simulink model "sm_car_"  (R2026b)
settings: Solver=ode23t  StopTime=100  MaxStep=0.4  AbsTol=1e-3  EnableMultiTasking=on
PreLoadFcn:
  | % Due to usability issue in Repeating Sequence block
  | warning('off','Simulink:Masking:Invalid');
  | 
  | % Eliminate unnecessary warnings in inactive variants
  | % Warnings generated only if you click through inactive variant
  | warning('off','MATLAB:nonExistentField');
  | warning('off','Simulink:Parameters:BlkParamUndefined');
PostLoadFcn:
  | set_param([bdroot '/Vehicle'],'popup_trailer','Off')
  | warning('off','sm:sli:setup:compile:LocalSolverNotSupported')
  | %sm_car_config_maneuver(bdroot,'WOT Braking');
  | sm_car_config_vehicle(bdroot,'false');
  | sm_car_config_logging(bdroot);
InitFcn:
  | sm_car_config_camera;
  | Vehicle = sm_car_vehcfg_checkConfig(Vehicle);
  | sm_car_check_tire_model(bdroot);
StartFcn:
  | tic;
StopFcn:
  | Elapsed_Sim_Time = toc;
  | % disp(['Elapsed Sim Time = ' num2str(Elapsed_Sim_Time)]);
undefined symbols (not defined in the file or in its folder): acc_theta, accel_ramp_rate, Axle1D, AxleIn, Camera, Control, Driver, Init, Maneuver, Pedal, Scene, ShaftL1, ShaftL2, ShaftR1, ShaftR2, Visual, X, xy_data_car_side, Y, Z
libraries: sm_lib x290, fl_lib x171, nesl_utility x144, simulink x60, simulink_extras x14, sdl_lib x14, SimscapeFluids_lib x7, Damper_Element x4, Tire_1x2x x4, ee_lib x3, Scene_Utilities x3, sharedTrackingLibrary x2
(part 3 of 22)

== system sm_car_/Camera Frames/Transform FR ==
  Transform Camera Frame : sm_lib/Frames and Transforms/Rigid Transform  RotationMethod=RotationSequence  FollAlignAxisA=+X  BaseAlignAxisA=+Y  FollAlignAxisB=+Y  BaseAlignAxisB=+Z  RotationStandardAxis=+Z  RotationAngle=0.0  RotationAngleUnits=deg  RotationArbitraryAxis=[0 0 1]  RotationSequenceAxes=FollowerAxes  RotationSequence=ZYX  RotationSequenceAngles=CF.a.Value(3:-1:1)  RotationSequenceAnglesUnits=deg  RotationMatrix=[1 0 0; 0 1 0; 0 0 1]  Quaternion=[1 0 0 0]  TranslationMethod=Cartesian  TranslationCartesianOffset=CF.s.Value  TranslationCartesianOffsetUnits=m  TranslationStandardAxis=+Z  TranslationStandardOffset=0  TranslationStandardOffsetUnits=m  TranslationROffset=0  TranslationROffsetUnits=m  TranslationThetaOffset=0  TranslationThetaOffsetUnits=deg  TranslationZOffset=0  TranslationZOffsetUnits=m
  B : PMIOPort  Side=Left
  F : PMIOPort  Port=2  Side=Right
  connections:
  Transform Camera Frame/RConn1 -- F/RConn1
  Transform Camera Frame/LConn1 -- B/RConn1

== system sm_car_/Camera Frames/Transform FixO FL ==
  Transform Camera Frame : sm_lib/Frames and Transforms/Rigid Transform  RotationMethod=RotationSequence  FollAlignAxisA=+X  BaseAlignAxisA=+Y  FollAlignAxisB=+Y  BaseAlignAxisB=+Z  RotationStandardAxis=+Z  RotationAngle=0.0  RotationAngleUnits=deg  RotationArbitraryAxis=[0 0 1]  RotationSequenceAxes=FollowerAxes  RotationSequence=ZYX  RotationSequenceAngles=CF.a.Value(3:-1:1)  RotationSequenceAnglesUnits=deg  RotationMatrix=[1 0 0; 0 1 0; 0 0 1]  Quaternion=[1 0 0 0]  TranslationMethod=Cartesian  TranslationCartesianOffset=CF.s.Value  TranslationCartesianOffsetUnits=m  TranslationStandardAxis=+Z  TranslationStandardOffset=0  TranslationStandardOffsetUnits=m  TranslationROffset=0  TranslationROffsetUnits=m  TranslationThetaOffset=0  TranslationThetaOffsetUnits=deg  TranslationZOffset=0  TranslationZOffsetUnits=m
  B : PMIOPort  Side=Left
  F : PMIOPort  Port=2  Side=Right
  connections:
  Transform Camera Frame/RConn1 -- F/RConn1
  Transform Camera Frame/LConn1 -- B/RConn1

== system sm_car_/Camera Frames/Transform FixO FR ==
  Transform Camera Frame : sm_lib/Frames and Transforms/Rigid Transform  RotationMethod=RotationSequence  FollAlignAxisA=+X  BaseAlignAxisA=+Y  FollAlignAxisB=+Y  BaseAlignAxisB=+Z  RotationStandardAxis=+Z  RotationAngle=0.0  RotationAngleUnits=deg  RotationArbitraryAxis=[0 0 1]  RotationSequenceAxes=FollowerAxes  RotationSequence=ZYX  RotationSequenceAngles=CF.a.Value(3:-1:1)  RotationSequenceAnglesUnits=deg  RotationMatrix=[1 0 0; 0 1 0; 0 0 1]  Quaternion=[1 0 0 0]  TranslationMethod=Cartesian  TranslationCartesianOffset=CF.s.Value  TranslationCartesianOffsetUnits=m  TranslationStandardAxis=+Z  TranslationStandardOffset=0  TranslationStandardOffsetUnits=m  TranslationROffset=0  TranslationROffsetUnits=m  TranslationThetaOffset=0  TranslationThetaOffsetUnits=deg  TranslationZOffset=0  TranslationZOffsetUnits=m
  B : PMIOPort  Side=Left
  F : PMIOPort  Port=2  Side=Right
  connections:
  Transform Camera Frame/RConn1 -- F/RConn1
  Transform Camera Frame/LConn1 -- B/RConn1

== system sm_car_/Camera Frames/Transform FixO Front ==
  Transform Camera Frame : sm_lib/Frames and Transforms/Rigid Transform  RotationMethod=RotationSequence  FollAlignAxisA=+X  BaseAlignAxisA=+Y  FollAlignAxisB=+Y  BaseAlignAxisB=+Z  RotationStandardAxis=+Z  RotationAngle=0.0  RotationAngleUnits=deg  RotationArbitraryAxis=[0 0 1]  RotationSequenceAxes=FollowerAxes  RotationSequence=ZYX  RotationSequenceAngles=CF.a.Value(3:-1:1)  RotationSequenceAnglesUnits=deg  RotationMatrix=[1 0 0; 0 1 0; 0 0 1]  Quaternion=[1 0 0 0]  TranslationMethod=Cartesian  TranslationCartesianOffset=CF.s.Value  TranslationCartesianOffsetUnits=m  TranslationStandardAxis=+Z  TranslationStandardOffset=0  TranslationStandardOffsetUnits=m  TranslationROffset=0  TranslationROffsetUnits=m  TranslationThetaOffset=0  TranslationThetaOffsetUnits=deg  TranslationZOffset=0  TranslationZOffsetUnits=m
  B : PMIOPort  Side=Left
  F : PMIOPort  Port=2  Side=Right
  connections:
  Transform Camera Frame/RConn1 -- F/RConn1
  Transform Camera Frame/LConn1 -- B/RConn1

== system sm_car_/Camera Frames/Transform FixO Left ==
  Transform Camera Frame : sm_lib/Frames and Transforms/Rigid Transform  RotationMethod=RotationSequence  FollAlignAxisA=+X  BaseAlignAxisA=+Y  FollAlignAxisB=+Y  BaseAlignAxisB=+Z  RotationStandardAxis=+Z  RotationAngle=0.0  RotationAngleUnits=deg  RotationArbitraryAxis=[0 0 1]  RotationSequenceAxes=FollowerAxes  RotationSequence=ZYX  RotationSequenceAngles=CF.a.Value(3:-1:1)  RotationSequenceAnglesUnits=deg  RotationMatrix=[1 0 0; 0 1 0; 0 0 1]  Quaternion=[1 0 0 0]  TranslationMethod=Cartesian  TranslationCartesianOffset=CF.s.Value  TranslationCartesianOffsetUnits=m  TranslationStandardAxis=+Z  TranslationStandardOffset=0  TranslationStandardOffsetUnits=m  TranslationROffset=0  TranslationROffsetUnits=m  TranslationThetaOffset=0  TranslationThetaOffsetUnits=deg  TranslationZOffset=0  TranslationZOffsetUnits=m
  B : PMIOPort  Side=Left
  F : PMIOPort  Port=2  Side=Right
  connections:
  Transform Camera Frame/RConn1 -- F/RConn1
  Transform Camera Frame/LConn1 -- B/RConn1

== system sm_car_/Camera Frames/Transform FixO RL ==
  Transform Camera Frame : sm_lib/Frames and Transforms/Rigid Transform  RotationMethod=RotationSequence  FollAlignAxisA=+X  BaseAlignAxisA=+Y  FollAlignAxisB=+Y  BaseAlignAxisB=+Z  RotationStandardAxis=+Z  RotationAngle=0.0  RotationAngleUnits=deg  RotationArbitraryAxis=[0 0 1]  RotationSequenceAxes=FollowerAxes  RotationSequence=ZYX  RotationSequenceAngles=CF.a.Value(3:-1:1)  RotationSequenceAnglesUnits=deg  RotationMatrix=[1 0 0; 0 1 0; 0 0 1]  Quaternion=[1 0 0 0]  TranslationMethod=Cartesian  TranslationCartesianOffset=CF.s.Value  TranslationCartesianOffsetUnits=m  TranslationStandardAxis=+Z  TranslationStandardOffset=0  TranslationStandardOffsetUnits=m  TranslationROffset=0  TranslationROffsetUnits=m  TranslationThetaOffset=0  TranslationThetaOffsetUnits=deg  TranslationZOffset=0  TranslationZOffsetUnits=m
  B : PMIOPort  Side=Left
  F : PMIOPort  Port=2  Side=Right
  connections:
  Transform Camera Frame/RConn1 -- F/RConn1
  Transform Camera Frame/LConn1 -- B/RConn1

== system sm_car_/Camera Frames/Transform FixO RR ==
  Transform Camera Frame : sm_lib/Frames and Transforms/Rigid Transform  RotationMethod=RotationSequence  FollAlignAxisA=+X  BaseAlignAxisA=+Y  FollAlignAxisB=+Y  BaseAlignAxisB=+Z  RotationStandardAxis=+Z  RotationAngle=0.0  RotationAngleUnits=deg  RotationArbitraryAxis=[0 0 1]  RotationSequenceAxes=FollowerAxes  RotationSequence=ZYX  RotationSequenceAngles=CF.a.Value(3:-1:1)  RotationSequenceAnglesUnits=deg  RotationMatrix=[1 0 0; 0 1 0; 0 0 1]  Quaternion=[1 0 0 0]  TranslationMethod=Cartesian  TranslationCartesianOffset=CF.s.Value  TranslationCartesianOffsetUnits=m  TranslationStandardAxis=+Z  TranslationStandardOffset=0  TranslationStandardOffsetUnits=m  TranslationROffset=0  TranslationROffsetUnits=m  TranslationThetaOffset=0  TranslationThetaOffsetUnits=deg  TranslationZOffset=0  TranslationZOffsetUnits=m
  B : PMIOPort  Side=Left
  F : PMIOPort  Port=2  Side=Right
  connections:
  Transform Camera Frame/RConn1 -- F/RConn1
  Transform Camera Frame/LConn1 -- B/RConn1

== system sm_car_/Camera Frames/Transform FixO Rear ==
  Transform Camera Frame : sm_lib/Frames and Transforms/Rigid Transform  RotationMethod=RotationSequence  FollAlignAxisA=+X  BaseAlignAxisA=+Y  FollAlignAxisB=+Y  BaseAlignAxisB=+Z  RotationStandardAxis=+Z  RotationAngle=0.0  RotationAngleUnits=deg  RotationArbitraryAxis=[0 0 1]  RotationSequenceAxes=FollowerAxes  RotationSequence=ZYX  RotationSequenceAngles=CF.a.Value(3:-1:1)  RotationSequenceAnglesUnits=deg  RotationMatrix=[1 0 0; 0 1 0; 0 0 1]  Quaternion=[1 0 0 0]  TranslationMethod=Cartesian  TranslationCartesianOffset=CF.s.Value  TranslationCartesianOffsetUnits=m  TranslationStandardAxis=+Z  TranslationStandardOffset=0  TranslationStandardOffsetUnits=m  TranslationROffset=0  TranslationROffsetUnits=m  TranslationThetaOffset=0  TranslationThetaOffsetUnits=deg  TranslationZOffset=0  TranslationZOffsetUnits=m
  B : PMIOPort  Side=Left
  F : PMIOPort  Port=2  Side=Right
  connections:
  Transform Camera Frame/RConn1 -- F/RConn1
  Transform Camera Frame/LConn1 -- B/RConn1

== system sm_car_/Camera Frames/Transform FixO Right ==
  Transform Camera Frame : sm_lib/Frames and Transforms/Rigid Transform  RotationMethod=RotationSequence  FollAlignAxisA=+X  BaseAlignAxisA=+Y  FollAlignAxisB=+Y  BaseAlignAxisB=+Z  RotationStandardAxis=+Z  RotationAngle=0.0  RotationAngleUnits=deg  RotationArbitraryAxis=[0 0 1]  RotationSequenceAxes=FollowerAxes  RotationSequence=ZYX  RotationSequenceAngles=CF.a.Value(3:-1:1)  RotationSequenceAnglesUnits=deg  RotationMatrix=[1 0 0; 0 1 0; 0 0 1]  Quaternion=[1 0 0 0]  TranslationMethod=Cartesian  TranslationCartesianOffset=CF.s.Value  TranslationCartesianOffsetUnits=m  TranslationStandardAxis=+Z  TranslationStandardOffset=0  TranslationStandardOffsetUnits=m  TranslationROffset=0  TranslationROffsetUnits=m  TranslationThetaOffset=0  TranslationThetaOffsetUnits=deg  TranslationZOffset=0  TranslationZOffsetUnits=m
  B : PMIOPort  Side=Left
  F : PMIOPort  Port=2  Side=Right
  connections:
  Transform Camera Frame/RConn1 -- F/RConn1
  Transform Camera Frame/LConn1 -- B/RConn1

== system sm_car_/Camera Frames/Transform FixO Top ==
  Transform Camera Frame : sm_lib/Frames and Transforms/Rigid Transform  RotationMethod=RotationSequence  FollAlignAxisA=+X  BaseAlignAxisA=+Y  FollAlignAxisB=+Y  BaseAlignAxisB=+Z  RotationStandardAxis=+Z  RotationAngle=0.0  RotationAngleUnits=deg  RotationArbitraryAxis=[0 0 1]  RotationSequenceAxes=FollowerAxes  RotationSequence=ZYX  RotationSequenceAngles=CF.a.Value(3:-1:1)  RotationSequenceAnglesUnits=deg  RotationMatrix=[1 0 0; 0 1 0; 0 0 1]  Quaternion=[1 0 0 0]  TranslationMethod=Cartesian  TranslationCartesianOffset=CF.s.Value  TranslationCartesianOffsetUnits=m  TranslationStandardAxis=+Z  TranslationStandardOffset=0  TranslationStandardOffsetUnits=m  TranslationROffset=0  TranslationROffsetUnits=m  TranslationThetaOffset=0  TranslationThetaOffsetUnits=deg  TranslationZOffset=0  TranslationZOffsetUnits=m
  B : PMIOPort  Side=Left
  F : PMIOPort  Port=2  Side=Right
  connections:
  Transform Camera Frame/RConn1 -- F/RConn1
  Transform Camera Frame/LConn1 -- B/RConn1

== system sm_car_/Camera Frames/Transform Front ==
  Transform Camera Frame : sm_lib/Frames and Transforms/Rigid Transform  RotationMethod=RotationSequence  FollAlignAxisA=+X  BaseAlignAxisA=+Y  FollAlignAxisB=+Y  BaseAlignAxisB=+Z  RotationStandardAxis=+Z  RotationAngle=0.0  RotationAngleUnits=deg  RotationArbitraryAxis=[0 0 1]  RotationSequenceAxes=FollowerAxes  RotationSequence=ZYX  RotationSequenceAngles=CF.a.Value(3:-1:1)  RotationSequenceAnglesUnits=deg  RotationMatrix=[1 0 0; 0 1 0; 0 0 1]  Quaternion=[1 0 0 0]  TranslationMethod=Cartesian  TranslationCartesianOffset=CF.s.Value  TranslationCartesianOffsetUnits=m  TranslationStandardAxis=+Z  TranslationStandardOffset=0  TranslationStandardOffsetUnits=m  TranslationROffset=0  TranslationROffsetUnits=m  TranslationThetaOffset=0  TranslationThetaOffsetUnits=deg  TranslationZOffset=0  TranslationZOffsetUnits=m
  B : PMIOPort  Side=Left
  F : PMIOPort  Port=2  Side=Right
  connections:
  Transform Camera Frame/RConn1 -- F/RConn1
  Transform Camera Frame/LConn1 -- B/RConn1

== system sm_car_/Camera Frames/Transform Left ==
  Transform Camera Frame : sm_lib/Frames and Transforms/Rigid Transform  RotationMethod=RotationSequence  FollAlignAxisA=+X  BaseAlignAxisA=+Y  FollAlignAxisB=+Y  BaseAlignAxisB=+Z  RotationStandardAxis=+Z  RotationAngle=0.0  RotationAngleUnits=deg  RotationArbitraryAxis=[0 0 1]  RotationSequenceAxes=FollowerAxes  RotationSequence=ZYX  RotationSequenceAngles=CF.a.Value(3:-1:1)  RotationSequenceAnglesUnits=deg  RotationMatrix=[1 0 0; 0 1 0; 0 0 1]  Quaternion=[1 0 0 0]  TranslationMethod=Cartesian  TranslationCartesianOffset=CF.s.Value  TranslationCartesianOffsetUnits=m  TranslationStandardAxis=+Z  TranslationStandardOffset=0  TranslationStandardOffsetUnits=m  TranslationROffset=0  TranslationROffsetUnits=m  TranslationThetaOffset=0  TranslationThetaOffsetUnits=deg  TranslationZOffset=0  TranslationZOffsetUnits=m
  B : PMIOPort  Side=Left
  F : PMIOPort  Port=2  Side=Right
  connections:
  Transform Camera Frame/RConn1 -- F/RConn1
  Transform Camera Frame/LConn1 -- B/RConn1

== system sm_car_/Camera Frames/Transform RL ==
  Transform Camera Frame : sm_lib/Frames and Transforms/Rigid Transform  RotationMethod=RotationSequence  FollAlignAxisA=+X  BaseAlignAxisA=+Y  FollAlignAxisB=+Y  BaseAlignAxisB=+Z  RotationStandardAxis=+Z  RotationAngle=0.0  RotationAngleUnits=deg  RotationArbitraryAxis=[0 0 1]  RotationSequenceAxes=FollowerAxes  RotationSequence=ZYX  RotationSequenceAngles=CF.a.Value(3:-1:1)  RotationSequenceAnglesUnits=deg  RotationMatrix=[1 0 0; 0 1 0; 0 0 1]  Quaternion=[1 0 0 0]  TranslationMethod=Cartesian  TranslationCartesianOffset=CF.s.Value  TranslationCartesianOffsetUnits=m  TranslationStandardAxis=+Z  TranslationStandardOffset=0  TranslationStandardOffsetUnits=m  TranslationROffset=0  TranslationROffsetUnits=m  TranslationThetaOffset=0  TranslationThetaOffsetUnits=deg  TranslationZOffset=0  TranslationZOffsetUnits=m
  B : PMIOPort  Side=Left
  F : PMIOPort  Port=2  Side=Right
  connections:
  Transform Camera Frame/RConn1 -- F/RConn1
  Transform Camera Frame/LConn1 -- B/RConn1

== system sm_car_/Camera Frames/Transform RR ==
  Transform Camera Frame : sm_lib/Frames and Transforms/Rigid Transform  RotationMethod=RotationSequence  FollAlignAxisA=+X  BaseAlignAxisA=+Y  FollAlignAxisB=+Y  BaseAlignAxisB=+Z  RotationStandardAxis=+Z  RotationAngle=0.0  RotationAngleUnits=deg  RotationArbitraryAxis=[0 0 1]  RotationSequenceAxes=FollowerAxes  RotationSequence=ZYX  RotationSequenceAngles=CF.a.Value(3:-1:1)  RotationSequenceAnglesUnits=deg  RotationMatrix=[1 0 0; 0 1 0; 0 0 1]  Quaternion=[1 0 0 0]  TranslationMethod=Cartesian  TranslationCartesianOffset=CF.s.Value  TranslationCartesianOffsetUnits=m  TranslationStandardAxis=+Z  TranslationStandardOffset=0  TranslationStandardOffsetUnits=m  TranslationROffset=0  TranslationROffsetUnits=m  TranslationThetaOffset=0  TranslationThetaOffsetUnits=deg  TranslationZOffset=0  TranslationZOffsetUnits=m
  B : PMIOPort  Side=Left
  F : PMIOPort  Port=2  Side=Right
  connections:
  Transform Camera Frame/RConn1 -- F/RConn1
  Transform Camera Frame/LConn1 -- B/RConn1

== system sm_car_/Camera Frames/Transform Rear ==
  Transform Camera Frame : sm_lib/Frames and Transforms/Rigid Transform  RotationMethod=RotationSequence  FollAlignAxisA=+X  BaseAlignAxisA=+Y  FollAlignAxisB=+Y  BaseAlignAxisB=+Z  RotationStandardAxis=+Z  RotationAngle=0.0  RotationAngleUnits=deg  RotationArbitraryAxis=[0 0 1]  RotationSequenceAxes=FollowerAxes  RotationSequence=ZYX  RotationSequenceAngles=CF.a.Value(3:-1:1)  RotationSequenceAnglesUnits=deg  RotationMatrix=[1 0 0; 0 1 0; 0 0 1]  Quaternion=[1 0 0 0]  TranslationMethod=Cartesian  TranslationCartesianOffset=CF.s.Value  TranslationCartesianOffsetUnits=m  TranslationStandardAxis=+Z  TranslationStandardOffset=0  TranslationStandardOffsetUnits=m  TranslationROffset=0  TranslationROffsetUnits=m  TranslationThetaOffset=0  TranslationThetaOffsetUnits=deg  TranslationZOffset=0  TranslationZOffsetUnits=m
  B : PMIOPort  Side=Left
  F : PMIOPort  Port=2  Side=Right
  connections:
  Transform Camera Frame/RConn1 -- F/RConn1
  Transform Camera Frame/LConn1 -- B/RConn1

== system sm_car_/Camera Frames/Transform Right ==
  Transform Camera Frame : sm_lib/Frames and Transforms/Rigid Transform  RotationMethod=RotationSequence  FollAlignAxisA=+X  BaseAlignAxisA=+Y  FollAlignAxisB=+Y  BaseAlignAxisB=+Z  RotationStandardAxis=+Z  RotationAngle=0.0  RotationAngleUnits=deg  RotationArbitraryAxis=[0 0 1]  RotationSequenceAxes=FollowerAxes  RotationSequence=ZYX  RotationSequenceAngles=CF.a.Value(3:-1:1)  RotationSequenceAnglesUnits=deg  RotationMatrix=[1 0 0; 0 1 0; 0 0 1]  Quaternion=[1 0 0 0]  TranslationMethod=Cartesian  TranslationCartesianOffset=CF.s.Value  TranslationCartesianOffsetUnits=m  TranslationStandardAxis=+Z  TranslationStandardOffset=0  TranslationStandardOffsetUnits=m  TranslationROffset=0  TranslationROffsetUnits=m  TranslationThetaOffset=0  TranslationThetaOffsetUnits=deg  TranslationZOffset=0  TranslationZOffsetUnits=m
  B : PMIOPort  Side=Left
  F : PMIOPort  Port=2  Side=Right
  connections:
  Transform Camera Frame/RConn1 -- F/RConn1
  Transform Camera Frame/LConn1 -- B/RConn1

== system sm_car_/Camera Frames/Transform SuspF ==
  Transform Camera Frame : sm_lib/Frames and Transforms/Rigid Transform  RotationMethod=RotationSequence  FollAlignAxisA=+X  BaseAlignAxisA=+Y  FollAlignAxisB=+Y  BaseAlignAxisB=+Z  RotationStandardAxis=+Z  RotationAngle=0.0  RotationAngleUnits=deg  RotationArbitraryAxis=[0 0 1]  RotationSequenceAxes=FollowerAxes  RotationSequence=ZYX  RotationSequenceAngles=CF.a.Value(3:-1:1)  RotationSequenceAnglesUnits=deg  RotationMatrix=[1 0 0; 0 1 0; 0 0 1]  Quaternion=[1 0 0 0]  TranslationMethod=Cartesian  TranslationCartesianOffset=CF.s.Value  TranslationCartesianOffsetUnits=m  TranslationStandardAxis=+Z  TranslationStandardOffset=0  TranslationStandardOffsetUnits=m  TranslationROffset=0  TranslationROffsetUnits=m  TranslationThetaOffset=0  TranslationThetaOffsetUnits=deg  TranslationZOffset=0  TranslationZOffsetUnits=m
  B : PMIOPort  Side=Left
  F : PMIOPort  Port=2  Side=Right
  connections:
  Transform Camera Frame/RConn1 -- F/RConn1
  Transform Camera Frame/LConn1 -- B/RConn1

== system sm_car_/Camera Frames/Transform SuspR ==
  Transform Camera Frame : sm_lib/Frames and Transforms/Rigid Transform  RotationMethod=RotationSequence  FollAlignAxisA=+X  BaseAlignAxisA=+Y  FollAlignAxisB=+Y  BaseAlignAxisB=+Z  RotationStandardAxis=+Z  RotationAngle=0.0  RotationAngleUnits=deg  RotationArbitraryAxis=[0 0 1]  RotationSequenceAxes=FollowerAxes  RotationSequence=ZYX  RotationSequenceAngles=CF.a.Value(3:-1:1)  RotationSequenceAnglesUnits=deg  RotationMatrix=[1 0 0; 0 1 0; 0 0 1]  Quaternion=[1 0 0 0]  TranslationMethod=Cartesian  TranslationCartesianOffset=CF.s.Value  TranslationCartesianOffsetUnits=m  TranslationStandardAxis=+Z  TranslationStandardOffset=0  TranslationStandardOffsetUnits=m  TranslationROffset=0  TranslationROffsetUnits=m  TranslationThetaOffset=0  TranslationThetaOffsetUnits=deg  TranslationZOffset=0  TranslationZOffsetUnits=m
  B : PMIOPort  Side=Left
  F : PMIOPort  Port=2  Side=Right
  connections:
  Transform Camera Frame/RConn1 -- F/RConn1
  Transform Camera Frame/LConn1 -- B/RConn1

== system sm_car_/Camera Frames/Transform Top ==
  Transform Camera Frame : sm_lib/Frames and Transforms/Rigid Transform  RotationMethod=RotationSequence  FollAlignAxisA=+X  BaseAlignAxisA=+Y  FollAlignAxisB=+Y  BaseAlignAxisB=+Z  RotationStandardAxis=+Z  RotationAngle=0.0  RotationAngleUnits=deg  RotationArbitraryAxis=[0 0 1]  RotationSequenceAxes=FollowerAxes  RotationSequence=ZYX  RotationSequenceAngles=CF.a.Value(3:-1:1)  RotationSequenceAnglesUnits=deg  RotationMatrix=[1 0 0; 0 1 0; 0 0 1]  Quaternion=[1 0 0 0]  TranslationMethod=Cartesian  TranslationCartesianOffset=CF.s.Value  TranslationCartesianOffsetUnits=m  TranslationStandardAxis=+Z  TranslationStandardOffset=0  TranslationStandardOffsetUnits=m  TranslationROffset=0  TranslationROffsetUnits=m  TranslationThetaOffset=0  TranslationThetaOffsetUnits=deg  TranslationZOffset=0  TranslationZOffsetUnits=m
  B : PMIOPort  Side=Left
  F : PMIOPort  Port=2  Side=Right
  connections:
  Transform Camera Frame/RConn1 -- F/RConn1
  Transform Camera Frame/LConn1 -- B/RConn1

== system sm_car_/Camera Frames/Transform View Seat FL ==
  Transform Camera Frame : sm_lib/Frames and Transforms/Rigid Transform  RotationMethod=RotationSequence  FollAlignAxisA=+X  BaseAlignAxisA=+Y  FollAlignAxisB=+Y  BaseAlignAxisB=+Z  RotationStandardAxis=+Z  RotationAngle=0.0  RotationAngleUnits=deg  RotationArbitraryAxis=[0 0 1]  RotationSequenceAxes=FollowerAxes  RotationSequence=ZYX  RotationSequenceAngles=CF.a.Value(3:-1:1)  RotationSequenceAnglesUnits=deg  RotationMatrix=[1 0 0; 0 1 0; 0 0 1]  Quaternion=[1 0 0 0]  TranslationMethod=Cartesian  TranslationCartesianOffset=CF.s.Value  TranslationCartesianOffsetUnits=m  TranslationStandardAxis=+Z  TranslationStandardOffset=0  TranslationStandardOffsetUnits=m  TranslationROffset=0  TranslationROffsetUnits=m  TranslationThetaOffset=0  TranslationThetaOffsetUnits=deg  TranslationZOffset=0  TranslationZOffsetUnits=m
  B : PMIOPort  Side=Left
  F : PMIOPort  Port=2  Side=Right
  connections:
  Transform Camera Frame/RConn1 -- F/RConn1
  Transform Camera Frame/LConn1 -- B/RConn1

== system sm_car_/Camera Frames/Transform View Seat FR ==
  Transform Camera Frame : sm_lib/Frames and Transforms/Rigid Transform  RotationMethod=RotationSequence  FollAlignAxisA=+X  BaseAlignAxisA=+Y  FollAlignAxisB=+Y  BaseAlignAxisB=+Z  RotationStandardAxis=+Z  RotationAngle=0.0  RotationAngleUnits=deg  RotationArbitraryAxis=[0 0 1]  RotationSequenceAxes=FollowerAxes  RotationSequence=ZYX  RotationSequenceAngles=CF.a.Value(3:-1:1)  RotationSequenceAnglesUnits=deg  RotationMatrix=[1 0 0; 0 1 0; 0 0 1]  Quaternion=[1 0 0 0]  TranslationMethod=Cartesian  TranslationCartesianOffset=CF.s.Value  TranslationCartesianOffsetUnits=m  TranslationStandardAxis=+Z  TranslationStandardOffset=0  TranslationStandardOffsetUnits=m  TranslationROffset=0  TranslationROffsetUnits=m  TranslationThetaOffset=0  TranslationThetaOffsetUnits=deg  TranslationZOffset=0  TranslationZOffsetUnits=m
  B : PMIOPort  Side=Left
  F : PMIOPort  Port=2  Side=Right
  connections:
  Transform Camera Frame/RConn1 -- F/RConn1
  Transform Camera Frame/LConn1 -- B/RConn1

== system sm_car_/Camera Frames/Transform View Susp FL ==
  Transform Camera Frame : sm_lib/Frames and Transforms/Rigid Transform  RotationMethod=RotationSequence  FollAlignAxisA=+X  BaseAlignAxisA=+Y  FollAlignAxisB=+Y  BaseAlignAxisB=+Z  RotationStandardAxis=+Z  RotationAngle=0.0  RotationAngleUnits=deg  RotationArbitraryAxis=[0 0 1]  RotationSequenceAxes=FollowerAxes  RotationSequence=ZYX  RotationSequenceAngles=CF.a.Value(3:-1:1)  RotationSequenceAnglesUnits=deg  RotationMatrix=[1 0 0; 0 1 0; 0 0 1]  Quaternion=[1 0 0 0]  TranslationMethod=Cartesian  TranslationCartesianOffset=CF.s.Value  TranslationCartesianOffsetUnits=m  TranslationStandardAxis=+Z  TranslationStandardOffset=0  TranslationStandardOffsetUnits=m  TranslationROffset=0  TranslationROffsetUnits=m  TranslationThetaOffset=0  TranslationThetaOffsetUnits=deg  TranslationZOffset=0  TranslationZOffsetUnits=m
  B : PMIOPort  Side=Left
  F : PMIOPort  Port=2  Side=Right
  connections:
  Transform Camera Frame/RConn1 -- F/RConn1
  Transform Camera Frame/LConn1 -- B/RConn1

== system sm_car_/Camera Frames/Transform View Susp FR ==
  Transform Camera Frame : sm_lib/Frames and Transforms/Rigid Transform  RotationMethod=RotationSequence  FollAlignAxisA=+X  BaseAlignAxisA=+Y  FollAlignAxisB=+Y  BaseAlignAxisB=+Z  RotationStandardAxis=+Z  RotationAngle=0.0  RotationAngleUnits=deg  RotationArbitraryAxis=[0 0 1]  RotationSequenceAxes=FollowerAxes  RotationSequence=ZYX  RotationSequenceAngles=CF.a.Value(3:-1:1)  RotationSequenceAnglesUnits=deg  RotationMatrix=[1 0 0; 0 1 0; 0 0 1]  Quaternion=[1 0 0 0]  TranslationMethod=Cartesian  TranslationCartesianOffset=CF.s.Value  TranslationCartesianOffsetUnits=m  TranslationStandardAxis=+Z  TranslationStandardOffset=0  TranslationStandardOffsetUnits=m  TranslationROffset=0  TranslationROffsetUnits=m  TranslationThetaOffset=0  TranslationThetaOffsetUnits=deg  TranslationZOffset=0  TranslationZOffsetUnits=m
  B : PMIOPort  Side=Left
  F : PMIOPort  Port=2  Side=Right
  connections:
  Transform Camera Frame/RConn1 -- F/RConn1
  Transform Camera Frame/LConn1 -- B/RConn1

== system sm_car_/Camera Frames/Transform View Susp RL ==
  Transform Camera Frame : sm_lib/Frames and Transforms/Rigid Transform  RotationMethod=RotationSequence  FollAlignAxisA=+X  BaseAlignAxisA=+Y  FollAlignAxisB=+Y  BaseAlignAxisB=+Z  RotationStandardAxis=+Z  RotationAngle=0.0  RotationAngleUnits=deg  RotationArbitraryAxis=[0 0 1]  RotationSequenceAxes=FollowerAxes  RotationSequence=ZYX  RotationSequenceAngles=CF.a.Value(3:-1:1)  RotationSequenceAnglesUnits=deg  RotationMatrix=[1 0 0; 0 1 0; 0 0 1]  Quaternion=[1 0 0 0]  TranslationMethod=Cartesian  TranslationCartesianOffset=CF.s.Value  TranslationCartesianOffsetUnits=m  TranslationStandardAxis=+Z  TranslationStandardOffset=0  TranslationStandardOffsetUnits=m  TranslationROffset=0  TranslationROffsetUnits=m  TranslationThetaOffset=0  TranslationThetaOffsetUnits=deg  TranslationZOffset=0  TranslationZOffsetUnits=m
  B : PMIOPort  Side=Left
  F : PMIOPort  Port=2  Side=Right
  connections:
  Transform Camera Frame/RConn1 -- F/RConn1
  Transform Camera Frame/LConn1 -- B/RConn1

== system sm_car_/Camera Frames/Transform View Susp RR ==
  Transform Camera Frame : sm_lib/Frames and Transforms/Rigid Transform  RotationMethod=RotationSequence  FollAlignAxisA=+X  BaseAlignAxisA=+Y  FollAlignAxisB=+Y  BaseAlignAxisB=+Z  RotationStandardAxis=+Z  RotationAngle=0.0  RotationAngleUnits=deg  RotationArbitraryAxis=[0 0 1]  RotationSequenceAxes=FollowerAxes  RotationSequence=ZYX  RotationSequenceAngles=CF.a.Value(3:-1:1)  RotationSequenceAnglesUnits=deg  RotationMatrix=[1 0 0; 0 1 0; 0 0 1]  Quaternion=[1 0 0 0]  TranslationMethod=Cartesian  TranslationCartesianOffset=CF.s.Value  TranslationCartesianOffsetUnits=m  TranslationStandardAxis=+Z  TranslationStandardOffset=0  TranslationStandardOffsetUnits=m  TranslationROffset=0  TranslationROffsetUnits=m  TranslationThetaOffset=0  TranslationThetaOffsetUnits=deg  TranslationZOffset=0  TranslationZOffsetUnits=m
  B : PMIOPort  Side=Left
  F : PMIOPort  Port=2  Side=Right
  connections:
  Transform Camera Frame/RConn1 -- F/RConn1
  Transform Camera Frame/LConn1 -- B/RConn1

== system sm_car_/Camera Frames/Transform Wheel FL ==
  Transform Camera Frame : sm_lib/Frames and Transforms/Rigid Transform  RotationMethod=RotationSequence  FollAlignAxisA=+X  BaseAlignAxisA=+Y  FollAlignAxisB=+Y  BaseAlignAxisB=+Z  RotationStandardAxis=+Z  RotationAngle=0.0  RotationAngleUnits=deg  RotationArbitraryAxis=[0 0 1]  RotationSequenceAxes=FollowerAxes  RotationSequence=ZYX  RotationSequenceAngles=CF.a.Value(3:-1:1)  RotationSequenceAnglesUnits=deg  RotationMatrix=[1 0 0; 0 1 0; 0 0 1]  Quaternion=[1 0 0 0]  TranslationMethod=Cartesian  TranslationCartesianOffset=CF.s.Value  TranslationCartesianOffsetUnits=m  TranslationStandardAxis=+Z  TranslationStandardOffset=0  TranslationStandardOffsetUnits=m  TranslationROffset=0  TranslationROffsetUnits=m  TranslationThetaOffset=0  TranslationThetaOffsetUnits=deg  TranslationZOffset=0  TranslationZOffsetUnits=m
  B : PMIOPort  Side=Left
  F : PMIOPort  Port=2  Side=Right
  connections:
  Transform Camera Frame/RConn1 -- F/RConn1
  Transform Camera Frame/LConn1 -- B/RConn1

== system sm_car_/Camera Frames/Transform Wheel FR ==
  Transform Camera Frame : sm_lib/Frames and Transforms/Rigid Transform  RotationMethod=RotationSequence  FollAlignAxisA=+X  BaseAlignAxisA=+Y  FollAlignAxisB=+Y  BaseAlignAxisB=+Z  RotationStandardAxis=+Z  RotationAngle=0.0  RotationAngleUnits=deg  RotationArbitraryAxis=[0 0 1]  RotationSequenceAxes=FollowerAxes  RotationSequence=ZYX  RotationSequenceAngles=CF.a.Value(3:-1:1)  RotationSequenceAnglesUnits=deg  RotationMatrix=[1 0 0; 0 1 0; 0 0 1]  Quaternion=[1 0 0 0]  TranslationMethod=Cartesian  TranslationCartesianOffset=CF.s.Value  TranslationCartesianOffsetUnits=m  TranslationStandardAxis=+Z  TranslationStandardOffset=0  TranslationStandardOffsetUnits=m  TranslationROffset=0  TranslationROffsetUnits=m  TranslationThetaOffset=0  TranslationThetaOffsetUnits=deg  TranslationZOffset=0  TranslationZOffsetUnits=m
  B : PMIOPort  Side=Left
  F : PMIOPort  Port=2  Side=Right
  connections:
  Transform Camera Frame/RConn1 -- F/RConn1
  Transform Camera Frame/LConn1 -- B/RConn1

== system sm_car_/Camera Frames/Transform Wheel RL ==
  Transform Camera Frame : sm_lib/Frames and Transforms/Rigid Transform  RotationMethod=RotationSequence  FollAlignAxisA=+X  BaseAlignAxisA=+Y  FollAlignAxisB=+Y  BaseAlignAxisB=+Z  RotationStandardAxis=+Z  RotationAngle=0.0  RotationAngleUnits=deg  RotationArbitraryAxis=[0 0 1]  RotationSequenceAxes=FollowerAxes  RotationSequence=ZYX  RotationSequenceAngles=CF.a.Value(3:-1:1)  RotationSequenceAnglesUnits=deg  RotationMatrix=[1 0 0; 0 1 0; 0 0 1]  Quaternion=[1 0 0 0]  TranslationMethod=Cartesian  TranslationCartesianOffset=CF.s.Value  TranslationCartesianOffsetUnits=m  TranslationStandardAxis=+Z  TranslationStandardOffset=0  TranslationStandardOffsetUnits=m  TranslationROffset=0  TranslationROffsetUnits=m  TranslationThetaOffset=0  TranslationThetaOffsetUnits=deg  TranslationZOffset=0  TranslationZOffsetUnits=m
  B : PMIOPort  Side=Left
  F : PMIOPort  Port=2  Side=Right
  connections:
  Transform Camera Frame/RConn1 -- F/RConn1
  Transform Camera Frame/LConn1 -- B/RConn1

== system sm_car_/Camera Frames/Transform Wheel RR ==
  Transform Camera Frame : sm_lib/Frames and Transforms/Rigid Transform  RotationMethod=RotationSequence  FollAlignAxisA=+X  BaseAlignAxisA=+Y  FollAlignAxisB=+Y  BaseAlignAxisB=+Z  RotationStandardAxis=+Z  RotationAngle=0.0  RotationAngleUnits=deg  RotationArbitraryAxis=[0 0 1]  RotationSequenceAxes=FollowerAxes  RotationSequence=ZYX  RotationSequenceAngles=CF.a.Value(3:-1:1)  RotationSequenceAnglesUnits=deg  RotationMatrix=[1 0 0; 0 1 0; 0 0 1]  Quaternion=[1 0 0 0]  TranslationMethod=Cartesian  TranslationCartesianOffset=CF.s.Value  TranslationCartesianOffsetUnits=m  TranslationStandardAxis=+Z  TranslationStandardOffset=0  TranslationStandardOffsetUnits=m  TranslationROffset=0  TranslationROffsetUnits=m  TranslationThetaOffset=0  TranslationThetaOffsetUnits=deg  TranslationZOffset=0  TranslationZOffsetUnits=m
  B : PMIOPort  Side=Left
  F : PMIOPort  Port=2  Side=Right
  connections:
  Transform Camera Frame/RConn1 -- F/RConn1
  Transform Camera Frame/LConn1 -- B/RConn1

== system sm_car_/Controller/Default ==
  DrvBus : Inport
  VehBus : Inport  Port=2
  Brake Control : Subsystem  Variant=on  VariantControlMode=label  VariantControl=Variant1  LabelModeActiveChoice=Pedal  mask{popup_brake_control=Pedal, abs_tire_radiusF=Vehicle.Chassis.Tire.tire_radius.Value, abs_tire_radiusR=Vehicle.Chassis.Tire.tire_radius.Value}
      mask prompts: popup_brake_control "Control Type"; abs_tire_radiusF "Tire Radius Front (m)"; abs_tire_radiusR "Tire Radius Rear (m)"
      mask init:
      | set_param(gcb,'LabelModeActiveChoice',get_param(gcb,'popup_brake_control'));
      settings: AttributesFormatString=%<ActiveVariant>
      mask TypeOptions popup_brake_control: Pedal | Pressure | ABS
      mask Display: disp(' ');
  Bus Creator1 : BusCreator  Inputs=4
  Bus Creator2 : BusCreator  Inputs=5
  Bus Selector : BusSelector  OutputSignals=Chassis.Body.CG.vx
  Bus Selector1 : BusSelector  OutputSignals=aSteerWheel,rAccelPedal,rBrakePedal
  Driveline Control : Subsystem
  Power Control : Subsystem  mask{trq_max=Control.Default.maxTrqRequest, trq_ratio_front=Control.Default.pcnt_torque_on_f, trq_rate_up=300, trq_rate_down=-5000}
      mask prompts: trq_max "Max Torque Request"; trq_ratio_front "Ratio of Torque on Front Wheels (0-1)"; trq_rate_up "Torque Rate Limit Up (N*m/s)"; trq_rate_down "Torque Rate Limit Down (N*m/s)"
  Spring Damper : Subsystem
  State Estimation : Subsystem
  Susp : Subsystem  mask{Steer=Control.Default.Steer}
      mask prompts: Steer "Steer (structure)"
  CtrlBus : Outport  VectorParamsAs1DForOutWhenUnconnected=off
  wires:
  DrvBus/1 -> Bus Selector1/1
  Bus Creator2/1 -> CtrlBus/1  "CtrlBus"
  Bus Selector1/2 -> Power Control/1(rAccelPedal)  "<rAccelPedal>"
  Spring Damper/2(Spring) -> Bus Creator1/4
  Power Control/1(Power) -> Bus Creator2/2
  Driveline Control/1(Driveline) -> Bus Creator2/3
  Spring Damper/1(Damper) -> Bus Creator1/3
  Bus Creator1/1 -> Bus Creator2/1  "Chassis"
  Brake Control/1(" Brakes") -> Bus Creator2/5
  Susp/1(SuspA1) -> Bus Creator1/1
  VehBus/1 -> Bus Selector/1, Power Control/2(VehBus), State Estimation/2(VehBus), Brake Control/2("VehBus ")
  Susp/2(SuspA2) -> Bus Creator1/2
  Bus Selector1/1 -> Susp/1(aSteerWheel), State Estimation/1(aSteerWheel)  "<aSteerWheel>"
  Bus Selector/1 -> Susp/2(vx)  "<vx>"
  State Estimation/1(StateEst) -> Power Control/3(StatesEst)
  Bus Selector1/3 -> [rBrakePedal]  "<rBrakePedal>"
  [rBrakePedal] -> Brake Control/1("rBrakePedal ")
  State Estimation/2(Meas) -> Bus Creator2/4  "Estimation"

== system sm_car_/Controller/FeedF_Ctrl ==
  DrvBus : Inport
  VehBus : Inport  Port=2
  Brake Control : Subsystem  Variant=on  VariantControlMode=label  VariantControl=Variant1  LabelModeActiveChoice=Pedal  mask{popup_brake_control=Pedal, abs_tire_radiusF=Vehicle.Chassis.TireA1.tire_radius.Value, abs_tire_radiusR=Vehicle.Chassis.TireA2.tire_radius.Value}
      mask prompts: popup_brake_control "Control Type"; abs_tire_radiusF "Tire Radius Front (m)"; abs_tire_radiusR "Tire Radius Rear (m)"
      mask init:
      | set_param(gcb,'LabelModeActiveChoice',get_param(gcb,'popup_brake_control'));
      settings: AttributesFormatString=%<ActiveVariant>
      mask TypeOptions popup_brake_control: Pedal | Pressure | ABS
      mask Display: disp(' ');
  Bus Creator1 : BusCreator  Inputs=4
  Bus Creator2 : BusCreator  Inputs=4
  Bus Selector : BusSelector  OutputSignals=Chassis.Body.CG.vx
  Bus Selector1 : BusSelector  OutputSignals=aSteerWheel,rAccelPedal,rBrakePedal
  Driveline Control : Subsystem
  Power Control : Subsystem  mask{Control=Control}
      mask prompts: Control "Control Parameters"
  Spring Damper : Subsystem
  Susp : Subsystem  mask{Steer=Control.Steer}
      mask prompts: Steer "Steer (structure)"
  CtrlBus : Outport  VectorParamsAs1DForOutWhenUnconnected=off
  wires:
  Bus Selector/1 -> Susp/2(vx)  "<vx>"
  Bus Selector1/1 -> Susp/1(aSteerWheel), Power Control/3(aSteerWheel)  "<aSteerWheel>"
  Susp/2(SuspA2) -> Bus Creator1/2
  VehBus/1 -> Bus Selector/1, Brake Control/2("VehBus "), Power Control/2(VehBus)
  Susp/1(SuspA1) -> Bus Creator1/1
  Brake Control/1(" Brakes") -> Bus Creator2/4
  Bus Creator1/1 -> Bus Creator2/1  "Chassis"
  Spring Damper/1(Damper) -> Bus Creator1/3
  Driveline Control/1(Driveline) -> Bus Creator2/3
  Power Control/1(Power) -> Bus Creator2/2  "Power"
  Spring Damper/2(Spring) -> Bus Creator1/4
  Bus Selector1/2 -> Power Control/1(rAccelPedal)  "<rAccelPedal>"
  Bus Selector1/3 -> Brake Control/1("rBrakePedal ")  "<rBrakePedal>"
  Bus Creator2/1 -> CtrlBus/1  "CtrlBus"
  DrvBus/1 -> Bus Selector1/1

== system sm_car_/Controller/NoIMU ==
  DrvBus : Inport
  VehBus : Inport  Port=2
  Brake Control : Subsystem  Variant=on  VariantControlMode=label  VariantControl=Variant1  LabelModeActiveChoice=Pedal  mask{popup_brake_control=Pedal, abs_tire_radiusF=Vehicle.Chassis.TireA1.tire_radius.Value, abs_tire_radiusR=Vehicle.Chassis.TireA2.tire_radius.Value}
      mask prompts: popup_brake_control "Control Type"; abs_tire_radiusF "Tire Radius Front (m)"; abs_tire_radiusR "Tire Radius Rear (m)"
      mask init:
      | set_param(gcb,'LabelModeActiveChoice',get_param(gcb,'popup_brake_control'));
      settings: AttributesFormatString=%<ActiveVariant>
      mask TypeOptions popup_brake_control: Pedal | Pressure | ABS
      mask Display: disp(' ');
  Bus Creator1 : BusCreator  Inputs=4
  Bus Creator2 : BusCreator  Inputs=4
  Bus Selector : BusSelector  OutputSignals=Chassis.Body.CG.vx
  Bus Selector1 : BusSelector  OutputSignals=aSteerWheel,rAccelPedal,rBrakePedal
  Driveline Control : Subsystem
  Power Control : Subsystem  mask(Control system parameters){Km=Control.NoIMU.CurrentTrqConst, Tmax=Control.NoIMU.Tmax, I0=Control.NoIMU.I0Load, w0=Control.NoIMU.wLoad, fis=Control.NoIMU.FuzzySystem}
      mask prompts: Km "Motor current-torque const"; Tmax "Max Torque"; I0 "No Load Current"; w0 "No Load RPM"; fis "Fuzzy System"
  Spring Damper : Subsystem
  Susp : Subsystem  mask{Steer=Control.Default.Steer}
      mask prompts: Steer "Steer (structure)"
  CtrlBus : Outport  VectorParamsAs1DForOutWhenUnconnected=off
  wires:
  Bus Selector/1 -> Susp/2(vx)  "<vx>"
  Bus Selector1/1 -> Susp/1(aSteerWheel)  "<aSteerWheel>"
  Susp/2(SuspA2) -> Bus Creator1/2
  VehBus/1 -> Bus Selector/1, Brake Control/2("VehBus "), Power Control/2(VehBus)
  Susp/1(SuspA1) -> Bus Creator1/1
  Brake Control/1(" Brakes") -> Bus Creator2/4
  Bus Creator1/1 -> Bus Creator2/1  "Chassis"
  Spring Damper/1(Damper) -> Bus Creator1/3
  Driveline Control/1(Driveline) -> Bus Creator2/3
  Power Control/1(Power) -> Bus Creator2/2
  Spring Damper/2(Spring) -> Bus Creator1/4
  Bus Selector1/2 -> Power Control/1(rAccelPedal)  "<rAccelPedal>"
  Bus Selector1/3 -> Brake Control/1("rBrakePedal ")  "<rBrakePedal>"
  Bus Creator2/1 -> CtrlBus/1  "CtrlBus"
  DrvBus/1 -> Bus Selector1/1

== system sm_car_/Controller/Slip_Ctrl ==
  DrvBus : Inport
  VehBus : Inport  Port=2
  Brake Control : Subsystem  Variant=on  VariantControlMode=label  VariantControl=Variant1  LabelModeActiveChoice=Pedal  mask{popup_brake_control=Pedal, abs_tire_radiusF=Vehicle.Chassis.Tire.tire_radius.Value, abs_tire_radiusR=Vehicle.Chassis.Tire.tire_radius.Value}
      mask prompts: popup_brake_control "Control Type"; abs_tire_radiusF "Tire Radius Front (m)"; abs_tire_radiusR "Tire Radius Rear (m)"
      mask init:
      | set_param(gcb,'LabelModeActiveChoice',get_param(gcb,'popup_brake_control'));
      settings: AttributesFormatString=%<ActiveVariant>
      mask TypeOptions popup_brake_control: Pedal | Pressure | ABS
      mask Display: disp(' ');
  Bus Creator1 : BusCreator  Inputs=4
  Bus Creator2 : BusCreator  Inputs=4
  Bus Selector : BusSelector  OutputSignals=Chassis.Body.CG.vx
  Bus Selector1 : BusSelector  OutputSignals=aSteerWheel,rAccelPedal,rBrakePedal
  Driveline Control : Subsystem
  Power Control : Subsystem  mask{Control=Control}
      mask prompts: Control "Control Parameters"
  Spring Damper : Subsystem
  Susp : Subsystem  mask{Steer=Control.Steer}
      mask prompts: Steer "Steer (structure)"
  CtrlBus : Outport  VectorParamsAs1DForOutWhenUnconnected=off
  wires:
  Bus Selector/1 -> Susp/2(vx)  "<vx>"
  Bus Selector1/1 -> Susp/1(aSteerWheel)  "<aSteerWheel>"
  Susp/2(SuspA2) -> Bus Creator1/2
  VehBus/1 -> Bus Selector/1, Power Control/2(VehBus), Brake Control/2("VehBus ")
  Susp/1(SuspA1) -> Bus Creator1/1
  Brake Control/1(" Brakes") -> Bus Creator2/4
  Bus Creator1/1 -> Bus Creator2/1  "Chassis"
  Spring Damper/1(Damper) -> Bus Creator1/3
  Driveline Control/1(Driveline) -> Bus Creator2/3
  Power Control/1(Power) -> Bus Creator2/2  "Power"
  Spring Damper/2(Spring) -> Bus Creator1/4
  Bus Selector1/2 -> Power Control/1(rAccelPedal)  "<rAccelPedal>"
  Bus Selector1/3 -> Brake Control/1("rBrakePedal ")  "<rBrakePedal>"
  Bus Creator2/1 -> CtrlBus/1  "CtrlBus"
  DrvBus/1 -> Bus Selector1/1

== system sm_car_/Controller/Slip_Ctrl_V2 ==
  DrvBus : Inport
  VehBus : Inport  Port=2
  Brake Control : Subsystem  Variant=on  VariantControlMode=label  VariantControl=Variant1  LabelModeActiveChoice=Pedal  mask{popup_brake_control=Pedal, abs_tire_radiusF=Vehicle.Chassis.Tire.tire_radius.Value, abs_tire_radiusR=Vehicle.Chassis.Tire.tire_radius.Value}
      mask prompts: popup_brake_control "Control Type"; abs_tire_radiusF "Tire Radius Front (m)"; abs_tire_radiusR "Tire Radius Rear (m)"
      mask init:
      | set_param(gcb,'LabelModeActiveChoice',get_param(gcb,'popup_brake_control'));
      settings: AttributesFormatString=%<ActiveVariant>
      mask TypeOptions popup_brake_control: Pedal | Pressure | ABS
      mask Display: disp(' ');
  Bus Creator1 : BusCreator  Inputs=4
  Bus Creator2 : BusCreator  Inputs=4
  Bus Selector : BusSelector  OutputSignals=Chassis.Body.CG.vx
  Bus Selector1 : BusSelector  OutputSignals=aSteerWheel,rAccelPedal,rBrakePedal
  Driveline Control : Subsystem
  Power Control : Subsystem  mask{Control=Control}
      mask prompts: Control "Control Parameters"
  Spring Damper : Subsystem
  Susp : Subsystem  mask{Steer=Control.Steer}
      mask prompts: Steer "Steer (structure)"
  CtrlBus : Outport  VectorParamsAs1DForOutWhenUnconnected=off
  wires:
  DrvBus/1 -> Bus Selector1/1
  Bus Creator2/1 -> CtrlBus/1  "CtrlBus"
  Bus Selector1/3 -> Brake Control/1("rBrakePedal ")  "<rBrakePedal>"
  Bus Selector1/2 -> Power Control/1(rAccelPedal)  "<rAccelPedal>"
  Spring Damper/2(Spring) -> Bus Creator1/4
  Power Control/1(Power) -> Bus Creator2/2  "Power"
  Driveline Control/1(Driveline) -> Bus Creator2/3
  Spring Damper/1(Damper) -> Bus Creator1/3
  Bus Creator1/1 -> Bus Creator2/1  "Chassis"
  Brake Control/1(" Brakes") -> Bus Creator2/4
  Susp/1(SuspA1) -> Bus Creator1/1
  VehBus/1 -> Power Control/2(VehBus), Brake Control/2("VehBus "), Bus Selector/1
  Susp/2(SuspA2) -> Bus Creator1/2
  Bus Selector1/1 -> Susp/1(aSteerWheel)  "<aSteerWheel>"
  Bus Selector/1 -> Susp/2(vx)  "<vx>"

== system sm_car_/Controller/TrqVec 4Motor ==
  DrvBus : Inport
  VehBus : Inport  Port=2
  Brake Control : Subsystem  Variant=on  VariantControlMode=label  VariantControl=Variant1  LabelModeActiveChoice=Pedal  mask{popup_brake_control=Pedal, abs_tire_radiusF=Vehicle.Chassis.TireA1.tire_radius.Value, abs_tire_radiusR=Vehicle.Chassis.TireA2.tire_radius.Value}
      mask prompts: popup_brake_control "Control Type"; abs_tire_radiusF "Tire Radius Front (m)"; abs_tire_radiusR "Tire Radius Rear (m)"
      mask init:
      | set_param(gcb,'LabelModeActiveChoice',get_param(gcb,'popup_brake_control'));
      settings: AttributesFormatString=%<ActiveVariant>
      mask TypeOptions popup_brake_control: Pedal | Pressure | ABS
      mask Display: disp(' ');
  Bus Creator1 : BusCreator  Inputs=4
  Bus Creator2 : BusCreator  Inputs=4
  Bus Selector : BusSelector  OutputSignals=aSteerWheel
  Bus Selector1 : BusSelector  OutputSignals=rBrakePedal
  Bus Selector2 : BusSelector  OutputSignals=Chassis.Body.CG.vx
  Driveline Control : Subsystem
  Power_TqVec : Subsystem  mask{Control=Control.TrqVec}
      mask prompts: Control "Control Parameters"
  Spring Damper : Subsystem
  Susp : Subsystem  mask{Steer=Control.Default.Steer}
      mask prompts: Steer "Steer (structure)"
  CtrlBus : Outport  VectorParamsAs1DForOutWhenUnconnected=off
  wires:
  Bus Selector2/1 -> Susp/2(vx)  "<vx>"
  Bus Selector/1 -> Susp/1(aSteerWheel)  "<aSteerWheel>"
  DrvBus/1 -> Bus Selector/1, Power_TqVec/1(DrvBus), Bus Selector1/1
  Bus Creator2/1 -> CtrlBus/1  "CtrlBus"
  Bus Selector1/1 -> Brake Control/1("rBrakePedal ")  "<rBrakePedal>"
  Spring Damper/2(Spring) -> Bus Creator1/4
  Power_TqVec/1(Power) -> Bus Creator2/2
  Driveline Control/1(Driveline) -> Bus Creator2/3
  Spring Damper/1(Damper) -> Bus Creator1/3
  Bus Creator1/1 -> Bus Creator2/1  "Chassis"
  Brake Control/1(" Brakes") -> Bus Creator2/4
  Susp/1(SuspA1) -> Bus Creator1/1
  VehBus/1 -> Brake Control/2("VehBus "), Power_TqVec/2(VehBus), Bus Selector2/1
  Susp/2(SuspA2) -> Bus Creator1/2

== system sm_car_/Controller/TrqVec_FLC ==
  DrvBus : Inport
  VehBus : Inport  Port=2
  Brake Control : Subsystem  Variant=on  VariantControlMode=label  VariantControl=Variant1  LabelModeActiveChoice=Pedal  mask{popup_brake_control=Pedal, abs_tire_radiusF=Vehicle.Chassis.Tire.tire_radius.Value, abs_tire_radiusR=Vehicle.Chassis.Tire.tire_radius.Value}
      mask prompts: popup_brake_control "Control Type"; abs_tire_radiusF "Tire Radius Front (m)"; abs_tire_radiusR "Tire Radius Rear (m)"
      mask init:
      | set_param(gcb,'LabelModeActiveChoice',get_param(gcb,'popup_brake_control'));
      settings: AttributesFormatString=%<ActiveVariant>
      mask TypeOptions popup_brake_control: Pedal | Pressure | ABS
      mask Display: disp(' ');
  Bus Creator1 : BusCreator  Inputs=4
  Bus Creator2 : BusCreator  Inputs=4
  Bus Selector : BusSelector  OutputSignals=Chassis.Body.CG.vx
  Bus Selector1 : BusSelector  OutputSignals=aSteerWheel,rAccelPedal,rBrakePedal
  Driveline Control : Subsystem
  Power Control : Subsystem  mask{Control=Control}
      mask prompts: Control "Control Parameters"
  Spring Damper : Subsystem
  Susp : Subsystem  mask{Steer=Control.Steer}
      mask prompts: Steer "Steer (structure)"
  CtrlBus : Outport  VectorParamsAs1DForOutWhenUnconnected=off
  wires:
  DrvBus/1 -> Bus Selector1/1
  Bus Creator2/1 -> CtrlBus/1  "CtrlBus"
  Bus Selector1/3 -> Brake Control/1("rBrakePedal ")  "<rBrakePedal>"
  Bus Selector1/2 -> Power Control/1(rAccelPedal)  "<rAccelPedal>"
  Spring Damper/2(Spring) -> Bus Creator1/4
  Power Control/1(Power) -> Bus Creator2/2  "Power"
  Driveline Control/1(Driveline) -> Bus Creator2/3
  Spring Damper/1(Damper) -> Bus Creator1/3
  Bus Creator1/1 -> Bus Creator2/1  "Chassis"
  Brake Control/1(" Brakes") -> Bus Creator2/4
  Susp/1(SuspA1) -> Bus Creator1/1
  VehBus/1 -> Power Control/2(VehBus), Brake Control/2("VehBus "), Bus Selector/1
  Susp/2(SuspA2) -> Bus Creator1/2
  Bus Selector1/1 -> Power Control/3(aSteerWheel), Susp/1(aSteerWheel)  "<aSteerWheel>"
  Bus Selector/1 -> Susp/2(vx)  "<vx>"

== system sm_car_/Controller/TrqVec_FLC_V2 ==
  DrvBus : Inport
  VehBus : Inport  Port=2
  Brake Control : Subsystem  Variant=on  VariantControlMode=label  VariantControl=Variant1  LabelModeActiveChoice=Pedal  mask{popup_brake_control=Pedal, abs_tire_radiusF=Vehicle.Chassis.Tire.tire_radius.Value, abs_tire_radiusR=Vehicle.Chassis.Tire.tire_radius.Value}
      mask prompts: popup_brake_control "Control Type"; abs_tire_radiusF "Tire Radius Front (m)"; abs_tire_radiusR "Tire Radius Rear (m)"
      mask init:
      | set_param(gcb,'LabelModeActiveChoice',get_param(gcb,'popup_brake_control'));
      settings: AttributesFormatString=%<ActiveVariant>
      mask TypeOptions popup_brake_control: Pedal | Pressure | ABS
      mask Display: disp(' ');
  Bus Creator1 : BusCreator  Inputs=4
  Bus Creator2 : BusCreator  Inputs=4
  Bus Selector : BusSelector  OutputSignals=Chassis.Body.CG.vx
  Bus Selector1 : BusSelector  OutputSignals=aSteerWheel,rAccelPedal,rBrakePedal
  Driveline Control : Subsystem
  Power Control : Subsystem  mask{Control=Control}
      mask prompts: Control "Control Parameters"
  Spring Damper : Subsystem
  Susp : Subsystem  mask{Steer=Control.Steer}
      mask prompts: Steer "Steer (structure)"
  CtrlBus : Outport  VectorParamsAs1DForOutWhenUnconnected=off
  wires:
  Bus Selector/1 -> Susp/2(vx)  "<vx>"
  Bus Selector1/1 -> Susp/1(aSteerWheel), Power Control/3(aSteerWheel)  "<aSteerWheel>"
  Susp/2(SuspA2) -> Bus Creator1/2
  VehBus/1 -> Bus Selector/1, Brake Control/2("VehBus "), Power Control/2(VehBus)
  Susp/1(SuspA1) -> Bus Creator1/1
  Brake Control/1(" Brakes") -> Bus Creator2/4
  Bus Creator1/1 -> Bus Creator2/1  "Chassis"
  Spring Damper/1(Damper) -> Bus Creator1/3
  Driveline Control/1(Driveline) -> Bus Creator2/3
  Power Control/1(Power) -> Bus Creator2/2  "Power"
  Spring Damper/2(Spring) -> Bus Creator1/4
  Bus Selector1/2 -> Power Control/1(rAccelPedal)  "<rAccelPedal>"
  Bus Selector1/3 -> Brake Control/1("rBrakePedal ")  "<rBrakePedal>"
  Bus Creator2/1 -> CtrlBus/1  "CtrlBus"
  DrvBus/1 -> Bus Selector1/1
